simulink model "Three_Stages"  (R2023a)
settings: Solver=FixedStepDiscrete  StartTime=0.0  StopTime=5000  FixedStep=1  RelTol=1e-3
values from neighbouring files (symbols this model uses):
  fw = zeros(16384, 1, 'uint32')    [test.m]
libraries: hdlsllib x27, simulink x27, etargetslib x1
(part 5 of 5)

== matlab function Three_Stages/MR/Subsystem/MATLAB Function ==
  data: state input uint8; next_state output; pending input uint16; cur_reg input uint8; processed input uint8; total input uint8; addr input uint32; base_reg_r input uint8; base_val input uint32; wb_r input boolean; is_load_r input boolean; is_push_r input boolean; ldrd_rt input uint8; ldrd_rt2 input uint8; rst_n input; start input; mr_op input; base input; base_reg input; reg_list input; rt input; rt2 input; wb input; next_pending output; next_cur_reg output; next_processed output; next_total output; next_addr output; next_base_reg_r output; next_base_val output; next_wb_r output; next_is_load_r output; next_is_push_r output; next_ldrd_rt output; next_ldrd_rt2 output
function [next_state, next_pending, next_cur_reg, next_processed, ...
          next_total, next_addr, next_base_reg_r, next_base_val, ...
          next_wb_r, next_is_load_r, next_is_push_r, ...
          next_ldrd_rt, next_ldrd_rt2] = mr_next_state( ...
    state, pending, cur_reg, processed, total, addr, base_reg_r, base_val, ...
    wb_r, is_load_r, is_push_r, ldrd_rt, ldrd_rt2, ...
    rst_n, start, mr_op, base, base_reg, reg_list, rt, rt2, wb)
%#codegen

% ---------- 状态编码 ----------
S_IDLE       = uint8(0);
S_SCAN       = uint8(1);
S_LOAD_REQ   = uint8(2);
S_LOAD_CAP   = uint8(3);
S_STORE_REQ  = uint8(5);
S_STORE_CAP  = uint8(6);
S_STOREW     = uint8(7);
S_BASE       = uint8(8);
S_LDRD_R1    = uint8(9);
S_LDRD_WB1   = uint8(10);
S_LDRD_R2    = uint8(11);
S_LDRD_WB2   = uint8(12);

% ---------- 显式声明所有输出变量的类型 ----------
next_state      = uint8(state);
next_pending    = uint16(pending);
next_cur_reg    = uint8(cur_reg);
next_processed  = uint8(processed);
next_total      = uint8(total);
next_addr       = uint32(addr);
next_base_reg_r = uint8(base_reg_r);
next_base_val   = uint32(base_val);
next_wb_r       = logical(wb_r);
next_is_load_r  = logical(is_load_r);
next_is_push_r  = logical(is_push_r);
next_ldrd_rt    = uint8(ldrd_rt);
next_ldrd_rt2   = uint8(ldrd_rt2);

% ---------- 复位 ----------
if rst_n == 0
    next_state = S_IDLE;
    next_pending = uint16(0);
    next_cur_reg = uint8(0);
    next_processed = uint8(0);
    next_total = uint8(0);
    next_addr = uint32(0);
    next_base_reg_r = uint8(0);
    next_base_val = uint32(0);
    next_wb_r = false;
    next_is_load_r = false;
    next_is_push_r = false;
    next_ldrd_rt = uint8(0);
    next_ldrd_rt2 = uint8(0);
    return;
end

% ---------- 状态转移 ----------
switch state
    case S_IDLE
        if start
            if mr_op == uint8(6)
                % LDRD 初始化
                next_state = S_LDRD_R1;
                next_ldrd_rt = uint8(rt);
                next_ldrd_rt2 = uint8(rt2);
                next_pending = uint16(0);
                next_total = uint8(2);
                next_addr = uint32(base);
                next_base_reg_r = uint8(base_reg);
                next_base_val = uint32(base);
                next_wb_r = logical(wb);
                next_is_load_r = false;
                next_is_push_r = false;
                next_processed = uint8(0);
            elseif reg_list ~= 0
                % LDM/STM/PUSH/POP 初始化
                next_state = S_SCAN;
                next_base_reg_r = uint8(base_reg);
                next_base_val = uint32(base);
                next_wb_r = logical(wb);
                next_is_load_r = (mr_op <= uint8(3));
                next_is_push_r = (mr_op == uint8(5));
                next_pending = uint16(reg_list);
                next_processed = uint8(0);
                
                total_temp = uint8(0);
                for k = 1:16
                    total_temp = total_temp + uint8(bitget(reg_list, k));
                end
                next_total = total_temp;
                
                if mr_op == uint8(5)
                    next_addr = uint32(base) - uint32(4) * uint32(total_temp);
                else
                    next_addr = uint32(base);
                end
            else
                % 单寄存器指令
                next_state = S_BASE;
                next_base_reg_r = uint8(base_reg);
                next_base_val = uint32(base);
                next_wb_r = logical(wb);
                next_is_push_r = (mr_op == uint8(5));
                next_processed = uint8(0);
                next_total = uint8(0);
            end
        else
            % ★★★ 关键新增：空闲状态下强制清零所有残留状态 ★★★
            next_state = S_IDLE;
            next_pending = uint16(0);
            next_cur_reg = uint8(0);
            next_processed = uint8(0);
            next_total = uint8(0);
            next_addr = uint32(0);       % 清空地址，防止 800016c 残留
            next_base_reg_r = uint8(0);
            next_base_val = uint32(0);
            next_wb_r = false;
            next_is_load_r = false;
            next_is_push_r = false;
            next_ldrd_rt = uint8(0);
            next_ldrd_rt2 = uint8(0);
        end

    case S_SCAN
        if pending == 0
            next_state = S_BASE;
        else
            low_bit = uint16(bitand(pending, bitcmp(pending - uint16(1))));
            cr = uint8(log2(double(low_bit)));
            next_cur_reg = cr;
            if is_load_r
                next_state = S_LOAD_REQ;
            else
                next_state = S_STORE_REQ;
            end
        end

    case S_LOAD_REQ
        next_state = S_LOAD_CAP;

    case S_LOAD_CAP
        next_pending = bitand(pending, bitcmp(bitshift(uint16(1), double(cur_reg))));
        next_processed = processed + uint8(1);
        next_addr = addr + uint32(4);
        
        if cur_reg == uint8(15)
            next_state = S_BASE;
            next_pending = uint16(0);
        else
            if (processed + uint8(1)) >= total
                next_state = S_BASE;
            else
                next_state = S_SCAN;
            end
        end

    case S_STORE_REQ
        next_state = S_STORE_CAP;

    case S_STORE_CAP
        next_state = S_STOREW;

    case S_STOREW
        next_pending = bitand(pending, bitcmp(bitshift(uint16(1), double(cur_reg))));
        next_processed = processed + uint8(1);
        next_addr = addr + uint32(4);
        
        if (processed + uint8(1)) >= total
            next_state = S_BASE;
        else
            next_state = S_SCAN;
        end

    case S_BASE
        next_state = S_IDLE;
        % 状态机退出前清理垃圾
        next_pending = uint16(0);
        next_processed = uint8(0);
        next_cur_reg = uint8(0);
        next_total = uint8(0);
        next_addr = uint32(0);
        next_base_val = uint32(0);
        next_is_load_r = false;
        next_is_push_r = false;
        next_ldrd_rt = uint8(0);
        next_ldrd_rt2 = uint8(0);

    case S_LDRD_R1
        next_state = S_LDRD_WB1;

    case S_LDRD_WB1
        next_state = S_LDRD_R2;
        next_addr = addr + uint32(4);

    case S_LDRD_R2
        next_state = S_LDRD_WB2;

    case S_LDRD_WB2
        next_state = S_IDLE;

    otherwise
        next_state = S_IDLE;
end
end
